simulink model "Bilanciamento_MPC_2024b"  (R2024b)
settings: Solver=FixedStepDiscrete  StartTime=0  StopTime=par_sim.t_fine  FixedStep=par_sim.Tint  RelTol=1e-3
PostLoadFcn:
  | % Path: la cartella di questo modello e le cartelle del progetto
  | % MPC_Range_Extension, due livelli sopra. La cartella del modello si
  | % aggiunge per ultima, cosi' ha la precedenza su altre versioni (v1.0).
  | cartella_modello  = fileparts(get_param('Bilanciamento_MPC', 'FileName'));
  | cartella_progetto = fileparts(fileparts(cartella_modello));
  | addpath(cartella_progetto, fullfile(cartella_progetto, 'modello'), fullfile(cartella_progetto, 'mpc'), fullfile(cartella_progetto, 'simulazione'), fullfile(cartella_progetto, 'grafici'));
  | addpath(cartella_modello);
  | clear cartella_modello cartella_progetto
  | 
  | % Parametri della simulazione, se non ci sono gia' (parametri_simulazione.m)
  | if ~evalin('base', 'exist(''par_sim'', ''var'')')
  |     assignin('base', 'par_sim', parametri_simulazione());
  | end
InitFcn:
  | % Path: la cartella di questo modello e le cartelle del progetto
  | % MPC_Range_Extension, due livelli sopra. La cartella del modello si
  | % aggiunge per ultima, cosi' ha la precedenza su altre versioni (v1.0).
  | cartella_modello  = fileparts(get_param('Bilanciamento_MPC', 'FileName'));
  | cartella_progetto = fileparts(fileparts(cartella_modello));
  | addpath(cartella_progetto, fullfile(cartella_progetto, 'modello'), fullfile(cartella_progetto, 'mpc'), fullfile(cartella_progetto, 'simulazione'), fullfile(cartella_progetto, 'grafici'));
  | addpath(cartella_modello);
  | clear cartella_modello cartella_progetto
  | 
  | % Parametri della simulazione, se non ci sono gia' (parametri_simulazione.m)
  | if ~evalin('base', 'exist(''par_sim'', ''var'')')
  |     assignin('base', 'par_sim', parametri_simulazione());
  | end
values from neighbouring files (symbols this model uses):
  par_sim = parametri_simulazione(par, pacco, formulazione, par.(['scenario' scenario]), orizzonte)    [avvio_simulink.m]    (also in simula_simulink.m = parametri_simulazione(par, pacco, tipo, scen, p))
libraries: simulink x2
settings Model: Creator=Acer  LastModifiedBy=Acer
settings ModelReferenceCC: UpdateModelReferenceTargets=IfOutOfDate
settings SFSimCC: SimGPUStackLimitPerThread=51200
settings RTWCC: GPUStackLimitPerThread=51200  GPUComputeCapability=7.5
settings ConfigComp: CovMetricSettings=de  CovBoundaryAbsTol=1.0e-5

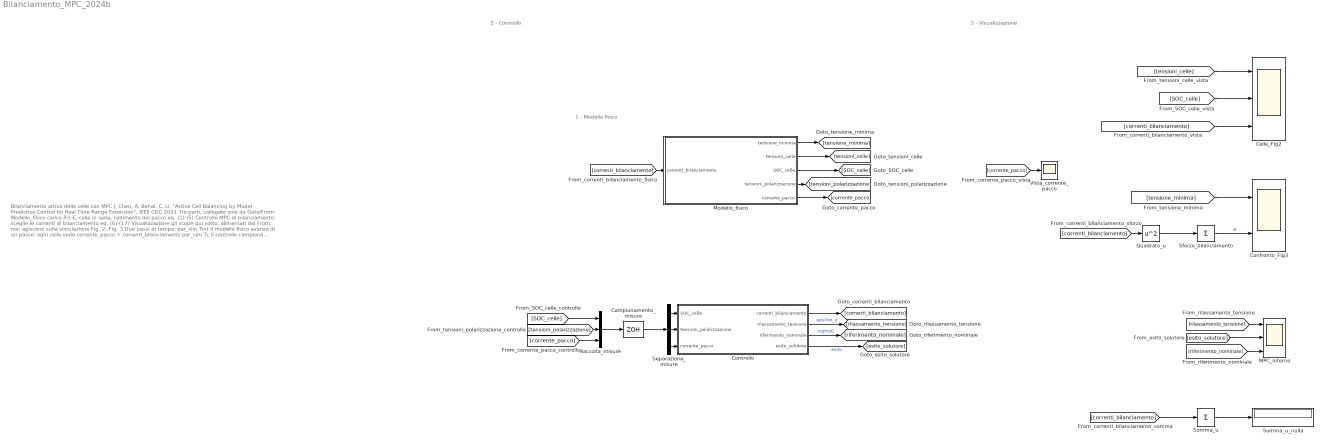
== system Bilanciamento_MPC_2024b ==
  note: Bilanciamento attivo delle celle con MPC
      | J. Chen, A. Behal, C. Li, "Active Cell Balancing by Model Predictive Control for Real Time Range Extension", IEEE CDC 2021
      |
      | Tre parti, collegate solo da Goto/From:
      |    Modello_fisico     carico R-L-E, celle in serie, cedimento del pacco             eq. (1)-(5)
      |    Controllo          MPC di bilanciamento: sceglie le correnti di bilanciamento    eq. (6)-(17)
      |    Visualizzazione    gli scope qui sotto, alimentati dai From: non agiscono sulla simulazione   Fig. 2, Fig. 3
      |
      | Due passi di tempo:
      |    par_sim.Tint         il modello fisico avanza di un passo: ogni cella vede corrente_pacco + correnti_bilanciamento
      |    par_sim.Tc           il controllo campiona corrente_pacco, SOC_celle e tensioni_polarizzazione e sceglie correnti_bilanciamento,
      |                         che restano costanti fino al passo di controllo successivo
      | La simulazione si ferma quando una cella scende sotto y_min.
      |
      | Parametri della simulazione nella struct 'par_sim' (avvio_simulink.m).
      | par_sim.n_J: 1 = J_t   2 = J_m   3 = J_Delta.  Confronto dei quattro casi: main_simulink.m
  note: 1 - Modello fisico
  note: 2 - Controllo
  note: 3 - Visualizzazione
  Campionamento_misure : ZeroOrderHold  SampleTime=par_sim.Tc
      settings: AttributesFormatString=ogni Tc
  Celle_Fig2 : Scope  NumInputPorts=3
      settings: AttributesFormatString=Fig. 2: y, s, u
  Confronto_Fig3 : Scope  NumInputPorts=2
      settings: AttributesFormatString=Fig. 3: min y, sforzo w
  Controllo : Subsystem
      settings: AttributesFormatString=MPC: problema (6) risolto\ncome QP (Remark 3)
  MPC_interno : Scope  NumInputPorts=3
      settings: AttributesFormatString=epsilon_y, esito, sigma0
  Modello_fisico : Subsystem
      settings: AttributesFormatString=carico, celle, cedimento\neq. (1)-(5)
  Quadrato_u : Math  Operator=square
  Raccolta_misure : Mux  Inputs=[par_sim.N par_sim.N 1]
  Separazione_misure : Demux  Outputs=[par_sim.N par_sim.N 1]
  Sforzo_bilanciamento : Sum  Inputs=+
  Somma_u : Sum  Inputs=+
      settings: AttributesFormatString=eq. (6f)
  Somma_u_nulla : Display
      settings: AttributesFormatString=deve restare 0
  Vista_corrente_pacco : Scope
  wires:
  [correnti_bilanciamento] -> Quadrato_u/1
  Quadrato_u/1 -> Sforzo_bilanciamento/1
  [correnti_bilanciamento] -> Somma_u/1
  [correnti_bilanciamento] -> Celle_Fig2/3
  [riferimento_nominale] -> MPC_interno/3
  [esito_solutore] -> MPC_interno/2
  [SOC_celle] -> Celle_Fig2/2
  [rilassamento_tensione] -> MPC_interno/1
  [tensioni_celle] -> Celle_Fig2/1
  Sforzo_bilanciamento/1 -> Confronto_Fig3/2  "w"
  [tensione_minima] -> Confronto_Fig3/1
  Somma_u/1 -> Somma_u_nulla/1
  Controllo/4(esito_solutore) -> [esito_solutore]  "esito"
  Controllo/3(riferimento_nominale) -> [riferimento_nominale]  "sigma0"
  Controllo/2(rilassamento_tensione) -> [rilassamento_tensione]  "epsilon_y"
  Controllo/1(correnti_bilanciamento) -> [correnti_bilanciamento]
  Modello_fisico/5(corrente_pacco) -> [corrente_pacco]
  Modello_fisico/4(tensioni_polarizzazione) -> [tensioni_polarizzazione]
  Modello_fisico/3(SOC_celle) -> [SOC_celle]
  Modello_fisico/2(tensioni_celle) -> [tensioni_celle]
  Modello_fisico/1(tensione_minima) -> [tensione_minima]
  [correnti_bilanciamento] -> Modello_fisico/1(correnti_bilanciamento)
  [corrente_pacco] -> Vista_corrente_pacco/1
  [tensioni_polarizzazione] -> Raccolta_misure/2
  [SOC_celle] -> Raccolta_misure/1
  [corrente_pacco] -> Raccolta_misure/3
  Raccolta_misure/1 -> Campionamento_misure/1
  Campionamento_misure/1 -> Separazione_misure/1
  Separazione_misure/3 -> Controllo/3(corrente_pacco)
  Separazione_misure/2 -> Controllo/2(tensioni_polarizzazione)
  Separazione_misure/1 -> Controllo/1(SOC_celle)

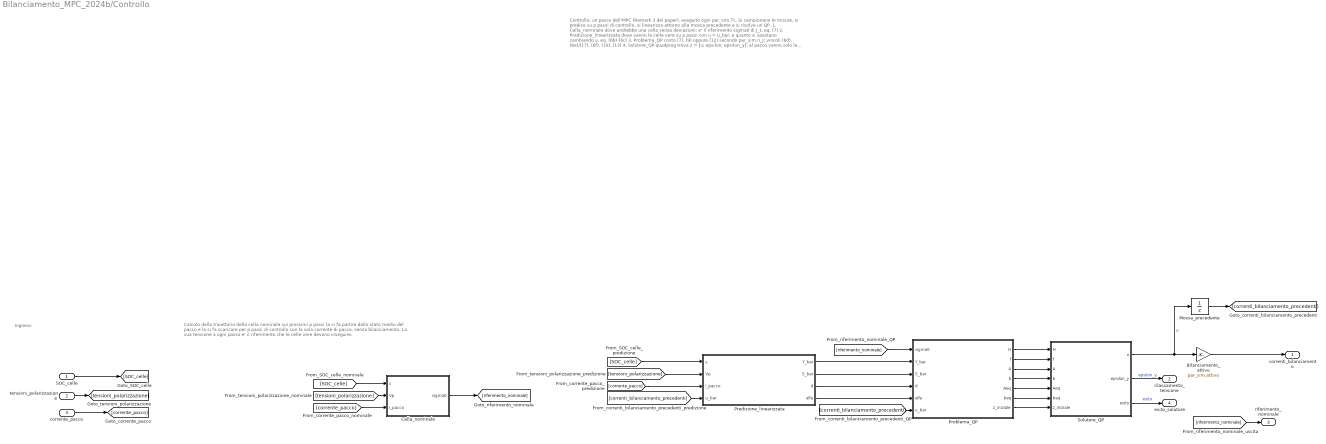
== system Bilanciamento_MPC_2024b/Controllo ==
  note: Ingressi
  note: Calcolo della traiettoria della cella nominale sui prossimi p passi
      |
      | la si fa partire dallo stato medio del pacco e la si fa scaricare per p passi di controllo con la sola corrente di pacco, senza bilanciamento.
      | La sua tensione a ogni passo e' il riferimento che le celle vere devono inseguire.
  note: Controllo: un passo dell'MPC (Remark 3 del paper), eseguito ogni par_sim.Tc. Si campionano le misure, si predice su p passi di controllo,
      | si linearizza attorno alla mossa precedente e si risolve un QP.
      |
      | 1. Cella_nominale            dove andrebbe una cella senza deviazioni: e' il riferimento sigma0 di J_t, eq. (7)
      | 2. Predizione_linearizzata   dove vanno le celle vere su p passi con u = u_bar, e quanto si spostano cambiando u, eq. (6b)-(6c)
      | 3. Problema_QP               costo (7), (9) oppure (12) secondo par_sim.n_J; vincoli (6d), (6e)/(17), (6f), (10), (13)
      | 4. Solutore_QP               quadprog trova z = [u; epsilon; epsilon_y]; al pacco vanno solo le u (orizzonte mobile)
      | 5. Bilanciamento_attivo      guadagno par_sim.attivo: con 0 il pacco lavora senza bilanciamento
      |
      | Doppio clic su un blocco per leggerne il codice: il calcolo e' tutto dentro il blocco.
  SOC_celle : Inport
  tensioni_polarizzazione : Inport  Port=2
  corrente_pacco : Inport  Port=3
  Bilanciamento_attivo : Gain  Gain=par_sim.attivo
      settings: AttributesFormatString=par_sim.attivo: 0 o 1
  Cella_nominale : MATLAB Function  TreatAsAtomicUnit=on
      settings: AttributesFormatString=eq. (7): riferimento sigma0
  Mossa_precedente : UnitDelay  InitialCondition=zeros(par_sim.N, 1)  SampleTime=par_sim.Tc
      settings: AttributesFormatString=u_bar = u_(k-1)
  Predizione_linearizzata : MATLAB Function  TreatAsAtomicUnit=on
      settings: AttributesFormatString=eq. (6b)-(6c), Remark 3
  Problema_QP : MATLAB Function  TreatAsAtomicUnit=on
      settings: AttributesFormatString=costo (7)/(9)/(12) e vincoli
  Solutore_QP : MATLAB Function  TreatAsAtomicUnit=on
      settings: AttributesFormatString=quadprog
  correnti_bilanciamento : Outport
  rilassamento_tensione : Outport  Port=2
  riferimento_nominale : Outport  Port=3
  esito_solutore : Outport  Port=4
  wires:
  corrente_pacco/1 -> [corrente_pacco]
  [corrente_pacco] -> Predizione_linearizzata/3(i_pacco)
  [tensioni_polarizzazione] -> Predizione_linearizzata/2(Vp)
  [SOC_celle] -> Predizione_linearizzata/1(s)
  [corrente_pacco] -> Cella_nominale/3(i_pacco)
  [tensioni_polarizzazione] -> Cella_nominale/2(Vp)
  [SOC_celle] -> Cella_nominale/1(s)
  Cella_nominale/1(sigma0) -> [riferimento_nominale]
  Predizione_linearizzata/1(Y_bar) -> Problema_QP/2(Y_bar)
  Predizione_linearizzata/2(S_bar) -> Problema_QP/3(S_bar)
  Predizione_linearizzata/3(d) -> Problema_QP/4(d)
  Predizione_linearizzata/4(alfa) -> Problema_QP/5(alfa)
  Problema_QP/1(H) -> Solutore_QP/1(H)
  Problema_QP/2(f) -> Solutore_QP/2(f)
  Problema_QP/3(A) -> Solutore_QP/3(A)
  Problema_QP/4(b) -> Solutore_QP/4(b)
  Problema_QP/5(Aeq) -> Solutore_QP/5(Aeq)
  Problema_QP/6(beq) -> Solutore_QP/6(beq)
  Problema_QP/7(z_iniziale) -> Solutore_QP/7(z_iniziale)
  [correnti_bilanciamento_precedenti] -> Predizione_linearizzata/4(u_bar)
  [correnti_bilanciamento_precedenti] -> Problema_QP/6(u_bar)
  Mossa_precedente/1 -> [correnti_bilanciamento_precedenti]
  Bilanciamento_attivo/1 -> correnti_bilanciamento/1
  Solutore_QP/1(u) -> Mossa_precedente/1, Bilanciamento_attivo/1  "u"
  tensioni_polarizzazione/1 -> [tensioni_polarizzazione]
  SOC_celle/1 -> [SOC_celle]
  [riferimento_nominale] -> riferimento_nominale/1
  [riferimento_nominale] -> Problema_QP/1(sigma0)
  Solutore_QP/2(epsilon_y) -> rilassamento_tensione/1  "epsilon_y"
  Solutore_QP/3(esito) -> esito_solutore/1  "esito"

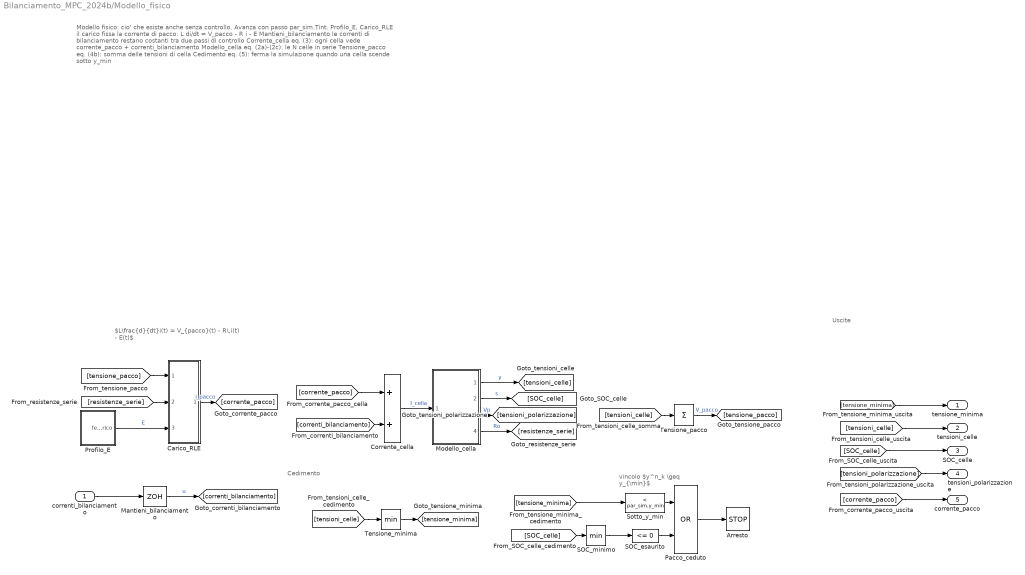
== system Bilanciamento_MPC_2024b/Modello_fisico ==
  note: vincolo $y^n_k \geq y_{\min}$
  note: $L\frac{d}{dt}i(t) = V_{pacco}(t) - R\,i(t) - E(t)$
  note: Cedimento
  note: Uscite
  note: Modello fisico: cio' che esiste anche senza controllo. Avanza con passo par_sim.Tint.
      |
      |    Profilo_E, Carico_RLE   il carico fissa la corrente di pacco:  L di/dt = V_pacco - R i - E
      |    Mantieni_bilanciamento  le correnti di bilanciamento restano costanti tra due passi di controllo
      |    Corrente_cella          eq. (3): ogni cella vede corrente_pacco + correnti_bilanciamento
      |    Modello_cella           eq. (2a)-(2c): le N celle in serie
      |    Tensione_pacco          eq. (4b): somma delle tensioni di cella
      |    Cedimento               eq. (5): ferma la simulazione quando una cella scende sotto y_min
  correnti_bilanciamento : Inport
  Arresto : Stop
  Carico_RLE : Subsystem
      settings: AttributesFormatString=L di_pacco/dt = V_pacco - R i_pacco - E
  Corrente_cella : Sum
      settings: AttributesFormatString=eq. (3): I_cella = i_pacco + u
  Mantieni_bilanciamento : ZeroOrderHold  SampleTime=par_sim.Tint
      settings: AttributesFormatString=costante tra due passi\ndi controllo
  Modello_cella : Subsystem
      settings: AttributesFormatString=eq. (2a)-(2c), (4a)
  Pacco_ceduto : Logic  Operator=OR  AllPortsSameDT=off  OutDataTypeStr=boolean
  Profilo_E : Subsystem
      settings: AttributesFormatString=f.e.m. del carico E(t)
  SOC_esaurito : simulink/Logic and Bit Operations/Compare To Constant  relop=<=  const=0  OutDataTypeStr=boolean
  SOC_minimo : MinMax
  Sotto_y_min : simulink/Logic and Bit Operations/Compare To Constant  relop=<  const=par_sim.y_min  OutDataTypeStr=boolean
  Tensione_minima : MinMax
  Tensione_pacco : Sum  Inputs=+
      settings: AttributesFormatString=eq. (4b)
  tensione_minima : Outport
  tensioni_celle : Outport  Port=2
  SOC_celle : Outport  Port=3
  tensioni_polarizzazione : Outport  Port=4
  corrente_pacco : Outport  Port=5
  wires:
  correnti_bilanciamento/1 -> Mantieni_bilanciamento/1
  [tensioni_celle] -> Tensione_pacco/1
  Modello_cella/1(tensioni_celle) -> [tensioni_celle]  "y"
  [correnti_bilanciamento] -> Corrente_cella/2
  [tensione_pacco] -> Carico_RLE/1(tensione_pacco)
  Modello_cella/2(SOC_celle) -> [SOC_celle]  "s"
  Tensione_pacco/1 -> [tensione_pacco]  "V_pacco"
  [resistenze_serie] -> Carico_RLE/2(resistenze_serie)
  Modello_cella/4(resistenze_serie) -> [resistenze_serie]  "Ro"
  Profilo_E/1(fem_carico) -> Carico_RLE/3(fem_carico)  "E"
  Corrente_cella/1 -> Modello_cella/1(correnti_celle)  "I_cella"
  Carico_RLE/1(corrente_pacco) -> [corrente_pacco]  "i_pacco"
  [corrente_pacco] -> Corrente_cella/1
  Mantieni_bilanciamento/1 -> [correnti_bilanciamento]  "u"
  [corrente_pacco] -> corrente_pacco/1
  [tensione_minima] -> tensione_minima/1
  [SOC_celle] -> SOC_celle/1
  Modello_cella/3(tensioni_polarizzazione) -> [tensioni_polarizzazione]  "Vp"
  [tensioni_polarizzazione] -> tensioni_polarizzazione/1
  [tensioni_celle] -> tensioni_celle/1
  Sotto_y_min/1 -> Pacco_ceduto/1
  [tensione_minima] -> Sotto_y_min/1
  SOC_minimo/1 -> SOC_esaurito/1
  Pacco_ceduto/1 -> Arresto/1
  [SOC_celle] -> SOC_minimo/1
  SOC_esaurito/1 -> Pacco_ceduto/2
  [tensioni_celle] -> Tensione_minima/1
  Tensione_minima/1 -> [tensione_minima]

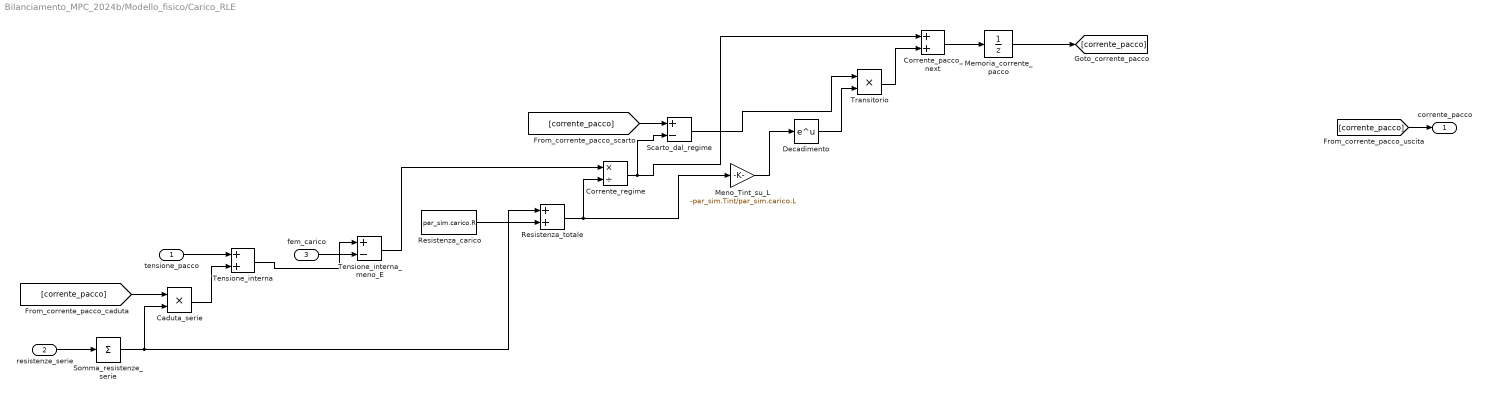
== system Bilanciamento_MPC_2024b/Modello_fisico/Carico_RLE ==
  tensione_pacco : Inport
  resistenze_serie : Inport  Port=2
  fem_carico : Inport  Port=3
  Caduta_serie : Product  Inputs=**
  Corrente_pacco_next : Sum
  Corrente_regime : Product  Inputs=*/
      settings: AttributesFormatString=(V_int - E) / R_tot
  Decadimento : Math
      settings: AttributesFormatString=exp(-Tint*R_tot/L)
  Memoria_corrente_pacco : UnitDelay  InitialCondition=par_sim.i_pacco_iniziale  SampleTime=par_sim.Tint
      settings: AttributesFormatString=stato i_pacco
  Meno_Tint_su_L : Gain  Gain=-par_sim.Tint/par_sim.carico.L
  Resistenza_carico : Constant  Value=par_sim.carico.R  SampleTime=par_sim.Tint
  Resistenza_totale : Sum
  Scarto_dal_regime : Sum  Inputs=+-
  Somma_resistenze_serie : Sum  Inputs=+
  Tensione_interna : Sum
      settings: AttributesFormatString=tensione del pacco a i_pacco = 0
  Tensione_interna_meno_E : Sum  Inputs=+-
  Transitorio : Product  Inputs=**
  corrente_pacco : Outport
  wires:
  [corrente_pacco] -> Scarto_dal_regime/1
  [corrente_pacco] -> Caduta_serie/1
  resistenze_serie/1 -> Somma_resistenze_serie/1
  Somma_resistenze_serie/1 -> Caduta_serie/2, Resistenza_totale/1
  Resistenza_carico/1 -> Resistenza_totale/2
  Memoria_corrente_pacco/1 -> [corrente_pacco]
  tensione_pacco/1 -> Tensione_interna/1
  Caduta_serie/1 -> Tensione_interna/2
  Tensione_interna/1 -> Tensione_interna_meno_E/1
  fem_carico/1 -> Tensione_interna_meno_E/2
  Tensione_interna_meno_E/1 -> Corrente_regime/1
  Resistenza_totale/1 -> Meno_Tint_su_L/1, Corrente_regime/2
  Meno_Tint_su_L/1 -> Decadimento/1
  Corrente_regime/1 -> Corrente_pacco_next/1, Scarto_dal_regime/2
  Scarto_dal_regime/1 -> Transitorio/1
  Decadimento/1 -> Transitorio/2
  Transitorio/1 -> Corrente_pacco_next/2
  Corrente_pacco_next/1 -> Memoria_corrente_pacco/1
  [corrente_pacco] -> corrente_pacco/1

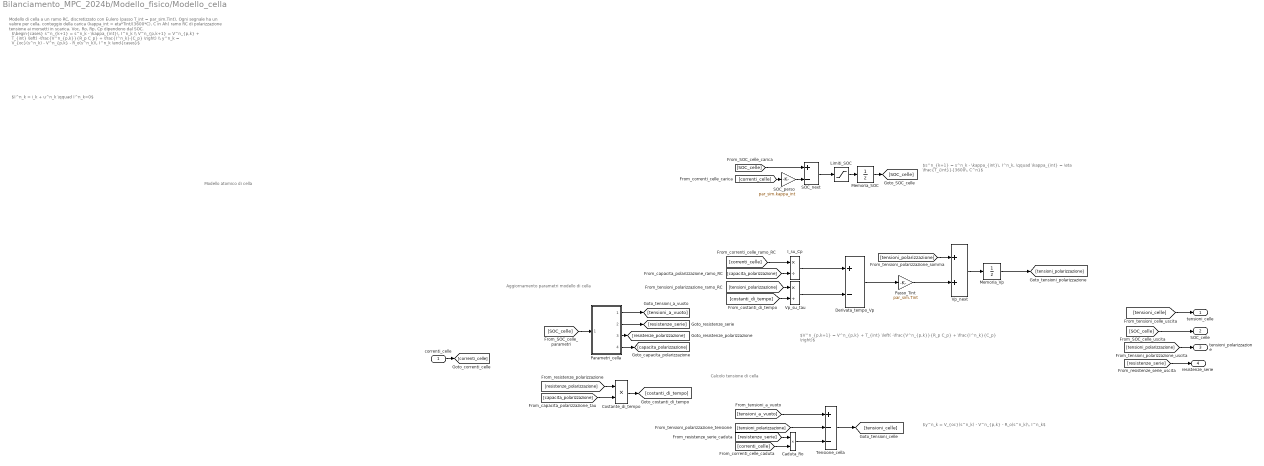
== system Bilanciamento_MPC_2024b/Modello_fisico/Modello_cella ==
  note: Modello atomico di cella
  note: $I^n_k = i_k + u^n_k \qquad I^n_k>0$
  note: $\begin{cases} s^n_{k+1} = s^n_k - \kappa_{int}\, I^n_k \\ V^n_{p,k+1} = V^n_{p,k} + T_{int} \left( -\frac{V^n_{p,k}}{R_p C_p} + \frac{I^n_k}{C_p} \right) \\ y^n_k = V_{oc}(s^n_k) - V^n_{p,k} - R_o(s^n_k)\, I^n_k \end{cases}$
  note: Calcolo tensione di cella
  note: Aggiornamento parametri modello di cella
  note: Modello di cella a un ramo RC, discretizzato con Eulero (passo T_int = par_sim.Tint). Ogni segnale ha un valore per cella.
      |
      | conteggio della carica (kappa_int = eta*Tint/(3600*C), C in Ah)
      |
      | ramo RC di polarizzazione
      |
      | tensione ai morsetti
      |
      | in scarica. Voc, Ro, Rp, Cp dipendono dal SOC.
  note: $V^n_{p,k+1} = V^n_{p,k} + T_{int} \left( -\frac{V^n_{p,k}}{R_p C_p} + \frac{I^n_k}{C_p} \right)$
  note: $y^n_k = V_{oc}(s^n_k) - V^n_{p,k} - R_o(s^n_k)\, I^n_k$
  note: $s^n_{k+1} = s^n_k - \kappa_{int}\, I^n_k, \qquad \kappa_{int} = \eta \frac{T_{int}}{3600\, C^n}$
  correnti_celle : Inport
  Caduta_Ro : Product  Inputs=**
  Costante_di_tempo : Product  Inputs=**
  Derivata_tempo_Vp : Sum  Inputs=+-
  I_su_Cp : Product  Inputs=*/
  Limiti_SOC : Saturate  UpperLimit=1  LowerLimit=0
  Memoria_SOC : UnitDelay  InitialCondition=par_sim.s_iniziale  SampleTime=par_sim.Tint
      settings: AttributesFormatString=stato s
  Memoria_Vp : UnitDelay  InitialCondition=par_sim.Vp_iniziale  SampleTime=par_sim.Tint
      settings: AttributesFormatString=stato V_p
  Parametri_cella : Subsystem
      settings: AttributesFormatString=V_oc, R_o, R_p, C_p(SOC)
  Passo_Tint : Gain  Gain=par_sim.Tint
  SOC_next : Sum  Inputs=+-
  SOC_perso : Gain  Gain=par_sim.kappa_int
      settings: AttributesFormatString=kappa_int * I_cella
  Tensione_cella : Sum  Inputs=+--
      settings: AttributesFormatString=eq. (2c)
  Vp_next : Sum
      settings: AttributesFormatString=eq. (2b)
  Vp_su_tau : Product  Inputs=*/
  tensioni_celle : Outport
  SOC_celle : Outport  Port=2
  tensioni_polarizzazione : Outport  Port=3
  resistenze_serie : Outport  Port=4
  wires:
  correnti_celle/1 -> [correnti_celle]
  [tensioni_polarizzazione] -> Vp_next/1
  [tensioni_polarizzazione] -> Vp_su_tau/1
  [tensioni_polarizzazione] -> Tensione_cella/2
  [SOC_celle] -> SOC_celle/1
  [SOC_celle] -> SOC_next/1
  [correnti_celle] -> I_su_Cp/1
  [correnti_celle] -> SOC_perso/1
  [correnti_celle] -> Caduta_Ro/2
  Vp_next/1 -> Memoria_Vp/1
  Passo_Tint/1 -> Vp_next/2
  Derivata_tempo_Vp/1 -> Passo_Tint/1
  Vp_su_tau/1 -> Derivata_tempo_Vp/2
  I_su_Cp/1 -> Derivata_tempo_Vp/1
  Limiti_SOC/1 -> Memoria_SOC/1
  SOC_next/1 -> Limiti_SOC/1
  SOC_perso/1 -> SOC_next/2
  Caduta_Ro/1 -> Tensione_cella/3
  Memoria_Vp/1 -> [tensioni_polarizzazione]
  Memoria_SOC/1 -> [SOC_celle]
  [SOC_celle] -> Parametri_cella/1(SOC_celle)
  [resistenze_serie] -> resistenze_serie/1
  [resistenze_serie] -> Caduta_Ro/1
  Parametri_cella/2(resistenze_serie) -> [resistenze_serie]
  [resistenze_polarizzazione] -> Costante_di_tempo/1
  Parametri_cella/3(resistenze_polarizzazione) -> [resistenze_polarizzazione]
  Parametri_cella/4(capacita_polarizzazione) -> [capacita_polarizzazione]
  [capacita_polarizzazione] -> Costante_di_tempo/2
  [capacita_polarizzazione] -> I_su_Cp/2
  [tensioni_a_vuoto] -> Tensione_cella/1
  Parametri_cella/1(tensioni_a_vuoto) -> [tensioni_a_vuoto]
  Costante_di_tempo/1 -> [costanti_di_tempo]
  [costanti_di_tempo] -> Vp_su_tau/2
  [tensioni_polarizzazione] -> tensioni_polarizzazione/1
  [tensioni_celle] -> tensioni_celle/1
  Tensione_cella/1 -> [tensioni_celle]

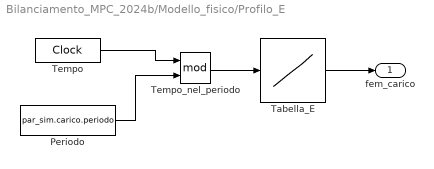
== system Bilanciamento_MPC_2024b/Modello_fisico/Profilo_E ==
  Periodo : Constant  Value=par_sim.carico.periodo  SampleTime=par_sim.Tint
  Tabella_E : Lookup_n-D  NumberOfTableDimensions=1  BreakpointsForDimension1=par_sim.carico.t_E  Table=par_sim.carico.E  ExtrapMethod=Clip  InternalRulePriority=Speed  RndMeth=Simplest
  Tempo : DigitalClock  SampleTime=par_sim.Tint
  Tempo_nel_periodo : Math  Operator=mod
  fem_carico : Outport
  wires:
  Tempo/1 -> Tempo_nel_periodo/1
  Periodo/1 -> Tempo_nel_periodo/2
  Tempo_nel_periodo/1 -> Tabella_E/1
  Tabella_E/1 -> fem_carico/1

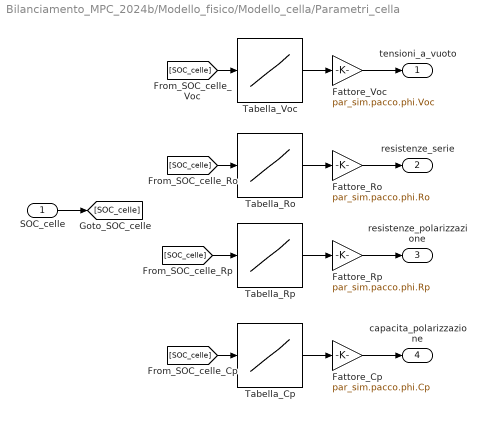
== system Bilanciamento_MPC_2024b/Modello_fisico/Modello_cella/Parametri_cella ==
  SOC_celle : Inport
  Fattore_Cp : Gain  Gain=par_sim.pacco.phi.Cp
  Fattore_Ro : Gain  Gain=par_sim.pacco.phi.Ro
  Fattore_Rp : Gain  Gain=par_sim.pacco.phi.Rp
  Fattore_Voc : Gain  Gain=par_sim.pacco.phi.Voc
  Tabella_Cp : Lookup_n-D  NumberOfTableDimensions=1  BreakpointsForDimension1=par_sim.pacco.s_tab  Table=par_sim.pacco.Cp_tab  ExtrapMethod=Clip  InternalRulePriority=Speed  RndMeth=Simplest
  Tabella_Ro : Lookup_n-D  NumberOfTableDimensions=1  BreakpointsForDimension1=par_sim.pacco.s_tab  Table=par_sim.pacco.Ro_tab  ExtrapMethod=Clip  InternalRulePriority=Speed  RndMeth=Simplest
  Tabella_Rp : Lookup_n-D  NumberOfTableDimensions=1  BreakpointsForDimension1=par_sim.pacco.s_tab  Table=par_sim.pacco.Rp_tab  ExtrapMethod=Clip  InternalRulePriority=Speed  RndMeth=Simplest
  Tabella_Voc : Lookup_n-D  NumberOfTableDimensions=1  BreakpointsForDimension1=par_sim.pacco.s_tab  Table=par_sim.pacco.Voc_tab  ExtrapMethod=Clip  InternalRulePriority=Speed  RndMeth=Simplest
  tensioni_a_vuoto : Outport
  resistenze_serie : Outport  Port=2
  resistenze_polarizzazione : Outport  Port=3
  capacita_polarizzazione : Outport  Port=4
  wires:
  Tabella_Voc/1 -> Fattore_Voc/1
  Tabella_Ro/1 -> Fattore_Ro/1
  Tabella_Rp/1 -> Fattore_Rp/1
  Tabella_Cp/1 -> Fattore_Cp/1
  Fattore_Voc/1 -> tensioni_a_vuoto/1
  Fattore_Ro/1 -> resistenze_serie/1
  Fattore_Rp/1 -> resistenze_polarizzazione/1
  Fattore_Cp/1 -> capacita_polarizzazione/1
  SOC_celle/1 -> [SOC_celle]
  [SOC_celle] -> Tabella_Rp/1
  [SOC_celle] -> Tabella_Cp/1
  [SOC_celle] -> Tabella_Voc/1
  [SOC_celle] -> Tabella_Ro/1

== matlab function Bilanciamento_MPC_2024b/Controllo/Predizione_linearizzata ==
  data: s input; Y_bar output; Vp input; i_pacco input; u_bar input; S_bar output; d output; alfa output; par_sim parameter
function [Y_bar, S_bar, d, alfa] = Predizione_linearizzata(s, Vp, i_pacco, u_bar, par_sim)
% PREDIZIONE LINEARIZZATA - eq. (6b)-(6c) del paper, linearizzate come nel
% Remark 3.
%
% Per ogni cella fa avanzare il modello per p passi di controllo, con la
% corrente di bilanciamento del passo precedente, e accanto a ogni
% equazione del modello calcola la sua derivata rispetto alla corrente.
% Con questi numeri la tensione e il SOC predetti diventano due rette
% nella corrente di bilanciamento u(n), [L, (6)]:
%
%   y(j,n) ~= Y_bar(j,n) + d(j,n)    * (u(n) - u_bar(n))
%   s(j,n) ~= S_bar(j,n) + alfa(j,n) * (u(n) - u_bar(n))
%
% Ingressi, all'istante k
%   s, Vp     SOC e tensione di polarizzazione misurati, N x 1
%   i_pacco   corrente di pacco misurata [A], positiva in scarica
%   u_bar     correnti di bilanciamento del passo precedente, N x 1
%   par_sim   parametri della simulazione (parametri_simulazione.m)
% Uscite, matrici p x N: riga j <-> istante k+j, colonna n <-> cella n
%   Y_bar, S_bar   tensione e SOC predetti con u = u_bar
%   d, alfa        coefficienti di sensibilita': di quanto cambiano la
%                  tensione [V/A] e il SOC [1/A] per ogni ampere in piu'
%
% Formule e numeri di equazione: Linearizzazione_MPC.pdf, citato [L].
% Le celle non si influenzano tra loro: si calcola una cella alla volta.

%% Dati
N  = par_sim.N;                         % numero di celle
p  = par_sim.p;                         % passi dell'orizzonte
Tc = par_sim.Tc;                        % [s] passo di controllo

% Tabelle nominali: ogni parametro in 7 punti di SOC, [L, sezione 2.2]
s_tab   = par_sim.pacco.s_tab;
Voc_tab = par_sim.pacco.Voc_tab;        % [V]   tensione a vuoto
Ro_tab  = par_sim.pacco.Ro_tab;         % [Ohm] resistenza serie
Rp_tab  = par_sim.pacco.Rp_tab;         % [Ohm] resistenza di polarizzazione
Cp_tab  = par_sim.pacco.Cp_tab;         % [F]   capacita' di polarizzazione

Y_bar = zeros(p, N);
S_bar = zeros(p, N);
d     = zeros(p, N);
alfa  = zeros(p, N);

%% Una cella alla volta
for n = 1:N

    % Parametri propri della cella n: ogni parametro e' la tabella nominale
    % per il fattore di deviazione phi della cella; kappa e' il SOC perso
    % in un passo per ogni ampere, [L, (5)]
    phi_Voc = par_sim.pacco.phi.Voc(n);
    phi_Ro  = par_sim.pacco.phi.Ro(n);
    phi_Rp  = par_sim.pacco.phi.Rp(n);
    phi_Cp  = par_sim.pacco.phi.Cp(n);
    kappa   = par_sim.pacco.kappa(n);

    % Punto di partenza: lo stato misurato. s_j e Vp_j contengono lo stato
    % della cella e vengono aggiornati a ogni passo: prima dell'aggiornamento
    % valgono all'istante k+j-1, dopo all'istante k+j.
    s_j  = s(n);
    Vp_j = Vp(n);

    % Corrente della cella nel punto di linearizzazione, costante su tutto
    % l'orizzonte, [L, (1)]
    I_cella = i_pacco + u_bar(n);

    % Derivate dello stato rispetto alla corrente: nulle all'istante k,
    % perche' lo stato misurato non dipende dalla corrente futura
    alfa_j = 0;                         % derivata del SOC
    beta_j = 0;                         % derivata della tensione di polarizzazione

    %% Un passo alla volta
    for j = 1:p

        % 1) Parametri del ramo RC e loro derivate rispetto al SOC, letti nel
        %    SOC di inizio passo
        [Rp, ds_Rp] = leggi_tabella(s_tab, Rp_tab, phi_Rp, s_j);
        [Cp, ds_Cp] = leggi_tabella(s_tab, Cp_tab, phi_Cp, s_j);
        tau    = Rp * Cp;                       % costante di tempo
        ds_tau = ds_Rp * Cp + Rp * ds_Cp;       % sua derivata rispetto al SOC

        % 2) Tensione di polarizzazione, [L, (3)], e sua derivata, [L, (7)].
        %    beta_j si aggiorna per prima, perche' usa Vp_j e alfa_j di
        %    inizio passo.
        beta_j = beta_j + Tc * ( -beta_j / tau ...                      % Vp dipende dalla corrente
                                 + Vp_j * ds_tau * alfa_j / tau^2 ...   % tau tramite il SOC
                                 + 1 / Cp ...                           % corrente diretta
                                 - I_cella * ds_Cp * alfa_j / Cp^2 );   % Cp tramite il SOC
        Vp_j   = Vp_j + Tc * (-Vp_j / tau + I_cella / Cp);

        % 3) SOC, [L, (2)], e sua derivata, [L, (8)]
        s_j    = s_j - kappa * I_cella;
        alfa_j = alfa_j - kappa;
        if s_j >= 1                     % una cella piena non si carica oltre
            s_j    = 1;
            alfa_j = 0;
        end

        % 4) Tensione ai morsetti, [L, (4)], e sua derivata, [L, (9)], con i
        %    parametri letti nel SOC di fine passo
        [Voc, ds_Voc] = leggi_tabella(s_tab, Voc_tab, phi_Voc, s_j);
        [Ro,  ds_Ro]  = leggi_tabella(s_tab, Ro_tab,  phi_Ro,  s_j);
        y   = Voc - Vp_j - Ro * I_cella;
        d_j = ds_Voc * alfa_j ...                   % Voc tramite il SOC
              - beta_j ...                          % Vp dipende dalla corrente
              - ds_Ro * alfa_j * I_cella ...        % Ro tramite il SOC
              - Ro;                                 % corrente diretta

        % 5) Riga j, colonna n delle quattro uscite
        Y_bar(j, n) = y;
        S_bar(j, n) = s_j;
        d(j, n)     = d_j;
        alfa(j, n)  = alfa_j;

    end
end

end


function [P, ds_P] = leggi_tabella(s_tab, P_tab, phi, s)
% Valore del parametro P nel SOC s e sua derivata rispetto al SOC, [L, (T)]:
%
%   P(s) = phi * ( P_tab(tratto) + m * (s - s_tab(tratto)) ),   ds_P = phi * m
%
% dove tratto e' il tratto della tabella che contiene s e m la sua
% pendenza. Fuori dalla tabella si usa il valore dell'estremo, con derivata
% nulla.

% SOC riportato dentro la tabella
s_limitato = min(max(s, s_tab(1)), s_tab(end));

% Tratto della tabella: s_tab(tratto) <= s_limitato < s_tab(tratto + 1).
% L'ultimo punto della tabella appartiene all'ultimo tratto.
tratto = 1;
for q = 2:numel(s_tab) - 1
    if s_limitato >= s_tab(q)
        tratto = q;
    end
end

% Pendenza del tratto, valore e derivata
m    = (P_tab(tratto + 1) - P_tab(tratto)) / (s_tab(tratto + 1) - s_tab(tratto));
P    = phi * (P_tab(tratto) + m * (s_limitato - s_tab(tratto)));
ds_P = phi * m;

if s < s_tab(1) || s > s_tab(end)       % fuori dalla tabella
    ds_P = 0;
end

end

== matlab function Bilanciamento_MPC_2024b/Controllo/Cella_nominale ==
  data: s input; sigma0 output; Vp input; i_pacco input; par_sim parameter
function sigma0 = Cella_nominale(s, Vp, i_pacco, par_sim)
% CELLA NOMINALE - riferimento sigma0 del costo J_t, eq. (7) del paper.
%
% Si prende una cella "ideale", con i parametri nominali (senza deviazioni),
% la si fa partire dallo stato medio del pacco e la si scarica per p passi
% di controllo con la sola corrente di pacco, senza bilanciamento. La sua
% tensione a ogni passo e' il riferimento che le celle vere devono
% inseguire. Le grandezze della cella nominale hanno il suffisso 0, come
% l'apice 0 del paper: s0, Vp0, y0.
%
% Ingressi, misurati all'istante k
%   s, Vp     SOC e tensione di polarizzazione di ogni cella, N x 1
%   i_pacco   corrente di pacco [A], positiva in scarica
%   par_sim   parametri della simulazione (parametri_simulazione.m)
% Uscita
%   sigma0    riferimento, p x 1: la riga j vale per l'istante k+j
%
% Il modello della cella e' quello di Linearizzazione_MPC.pdf, citato [L]:
% equazioni (2), (3) e (4).

%% Dati
p     = par_sim.p;                      % passi dell'orizzonte
Tc    = par_sim.Tc;                     % [s] passo di controllo
kappa = par_sim.nominale.kappa;         % SOC perso in un passo per ogni ampere, [L, (5)]

% Tabelle della cella nominale: ogni parametro in 7 punti di SOC
s_tab   = par_sim.nominale.s_tab;
Voc_tab = par_sim.nominale.Voc_tab;     % [V]   tensione a vuoto
Ro_tab  = par_sim.nominale.Ro_tab;      % [Ohm] resistenza serie
Rp_tab  = par_sim.nominale.Rp_tab;      % [Ohm] resistenza di polarizzazione
Cp_tab  = par_sim.nominale.Cp_tab;      % [F]   capacita' di polarizzazione

%% Stato di partenza: la media delle celle del pacco
s0  = mean(s);
Vp0 = mean(Vp);

%% Scarica della cella nominale, un passo alla volta
sigma0 = zeros(p, 1);

for j = 1:p

    % Parametri del ramo RC nel SOC di inizio passo. Le tabelle vanno da
    % SOC 0 a SOC 1: fuori si usa il valore dell'estremo.
    s_limitato = min(max(s0, s_tab(1)), s_tab(end));
    Rp = interp1(s_tab, Rp_tab, s_limitato);
    Cp = interp1(s_tab, Cp_tab, s_limitato);

    % [L, (3)] tensione di polarizzazione a fine passo
    Vp0 = Vp0 + Tc * (-Vp0 / (Rp * Cp) + i_pacco / Cp);

    % [L, (2)] SOC a fine passo; una cella piena non si carica oltre
    s0 = s0 - kappa * i_pacco;
    if s0 > 1
        s0 = 1;
    end

    % [L, (4)] tensione ai morsetti a fine passo, con i parametri letti nel
    % nuovo SOC
    s_limitato = min(max(s0, s_tab(1)), s_tab(end));
    Voc = interp1(s_tab, Voc_tab, s_limitato);
    Ro  = interp1(s_tab, Ro_tab,  s_limitato);
    y0  = Voc - Vp0 - Ro * i_pacco;

    % Grandezza inseguita: la tensione, come nel paper, oppure il SOC
    if par_sim.sigma_tensione == 1
        sigma0(j) = y0;
    else
        sigma0(j) = s0;
    end

end

end

== matlab function Bilanciamento_MPC_2024b/Controllo/Problema_QP ==
  data: sigma0 input; H output; Y_bar input; S_bar input; d input; alfa input; u_bar input; f output; A output; b output; Aeq output; beq output; z_iniziale output; par_sim parameter
function [H, f, A, b, Aeq, beq, z_iniziale] = Problema_QP(sigma0, Y_bar, S_bar, d, alfa, u_bar, par_sim)
% PROBLEMA QP - il problema (6) del paper scritto come problema quadratico
% (Remark 3), nella forma che quadprog sa risolvere:
%
%   min  1/2*z'*H*z + f'*z     con  A*z <= b  e  Aeq*z = beq
%
% Il blocco non risolve nulla: riempie le matrici, un elemento alla volta,
% seguendo la procedura della sezione 8 di Problema_QP_MPC.pdf, citato [Q].
% I numeri come [Q, (12)] sono le equazioni di quel documento.
%
% Ingressi
%   sigma0         riferimento della cella nominale, p x 1 (serve solo a J_t)
%   Y_bar, S_bar   tensione e SOC predetti con u = u_bar, p x N
%   d, alfa        coefficienti di sensibilita' di tensione e SOC, p x N
%   u_bar          correnti di bilanciamento del passo precedente, N x 1
%   par_sim        parametri della simulazione (parametri_simulazione.m)
% Uscite
%   H, f, A, b, Aeq, beq   dati del QP
%   z_iniziale             punto di partenza ammissibile per quadprog
% Nelle matrici p x N la riga j corrisponde all'istante k+j, la colonna n
% alla cella n.

%% Dati
N     = par_sim.N;              % numero di celle
p     = par_sim.p;              % passi dell'orizzonte
n_J   = par_sim.n_J;            % formulazione: 1 = J_t, 2 = J_m, 3 = J_Delta
rho   = par_sim.rho;            % peso sulle correnti di bilanciamento
W     = par_sim.W;              % peso sulla variabile epsilon_y
y_min = par_sim.y_min;          % [V] tensione minima di cella
u_min = par_sim.u_min;          % [A] limiti della corrente di bilanciamento
u_max = par_sim.u_max;          % [A]

%% Incognite z = [u; epsilon; epsilon_y], [Q, sezione 8.1]
%   u(n)           corrente di bilanciamento della cella n     posizione n
%   epsilon(j)     minorante al passo j (J_m e J_Delta)        posizione N + j
%   epsilon(p+j)   maggiorante al passo j (solo J_Delta)       posizione N + p + j
%   epsilon_y      rilassamento della tensione minima          ultima posizione
n_z   = N + (n_J - 1) * p + 1;          % numero di incognite, [Q, (25)]
n_dis = n_J * p * N + 2 * N + 1;        % numero di vincoli di disuguaglianza, [Q, (25)]
pos_epsilon_y = n_z;                    % posizione di epsilon_y

%% Predizione linearizzata, [Q, (9)]
% Con la corrente u(n) la tensione predetta e'
%   y(j,n) = Y_lib(j,n) + d(j,n) * u(n)
% Y_lib e' la risposta libera: la tensione che si avrebbe senza bilanciamento.
Y_lib = zeros(p, N);
for n = 1:N
    for j = 1:p
        Y_lib(j, n) = Y_bar(j, n) - d(j, n) * u_bar(n);
    end
end

% Grandezza bilanciata sigma, usata dal costo e dai vincoli sulle epsilon:
% la tensione, come nel progetto, oppure il SOC ([Q, sezione 11]). Il
% vincolo di tensione minima usa sempre la tensione.
if par_sim.sigma_tensione == 1
    Sigma_bar = Y_bar;
    d_sigma   = d;
else
    Sigma_bar = S_bar;
    d_sigma   = alfa;
end
Sigma_lib = zeros(p, N);
for n = 1:N
    for j = 1:p
        Sigma_lib(j, n) = Sigma_bar(j, n) - d_sigma(j, n) * u_bar(n);
    end
end

%% Costruzione di H e di f, [Q, sezione 8.2]
H = zeros(n_z, n_z);
f = zeros(n_z, 1);

% Passo 1 - penalita' W*epsilon_y^2 (tutte le formulazioni), [Q, (13)]
H(pos_epsilon_y, pos_epsilon_y) = 2 * W;

% Passo 2 - peso rho*u(n)^2 sulle correnti (tutte le formulazioni), [Q, (14)]
for n = 1:N
    H(n, n) = 2 * rho;
end

% Passo 3 - inseguimento della cella nominale (solo J_t), [Q, (15)]
if n_J == 1
    for n = 1:N
        somma_d2 = 0;           % somma sui passi di d(j,n)^2
        somma_dc = 0;           % somma sui passi di d(j,n) * (Y_lib(j,n) - sigma0(j))
        for j = 1:p
            somma_d2 = somma_d2 + d_sigma(j, n)^2;
            somma_dc = somma_dc + d_sigma(j, n) * (Sigma_lib(j, n) - sigma0(j));
        end
        H(n, n) = H(n, n) + 2 * somma_d2;
        f(n)    = 2 * somma_dc;
    end
end

% Passo 4 - minoranti: nel costo -epsilon(j) (J_m e J_Delta), [Q, (18)]
if n_J == 2 || n_J == 3
    for j = 1:p
        f(N + j) = -1;
    end
end

% Passo 5 - maggioranti: nel costo +epsilon(p+j) (solo J_Delta), [Q, (21)]
if n_J == 3
    for j = 1:p
        f(N + p + j) = 1;
    end
end

%% Costruzione di A e di b, [Q, sezione 8.3]
% Ogni vincolo occupa una riga nuova: q e' il numero dell'ultima riga scritta.
A = zeros(n_dis, n_z);
b = zeros(n_dis, 1);
q = 0;

% Blocco 1 - tensione minima (tutte le formulazioni), [Q, (12)]:
%   -d(j,n)*u(n) - epsilon_y <= Y_lib(j,n) - y_min
for n = 1:N
    for j = 1:p
        q = q + 1;
        A(q, n)             = -d(j, n);
        A(q, pos_epsilon_y) = -1;
        b(q)                = Y_lib(j, n) - y_min;
    end
end

% Blocco 2 - minoranti (J_m e J_Delta), [Q, (17)]:
%   -d(j,n)*u(n) + epsilon(j) <= Y_lib(j,n)
if n_J == 2 || n_J == 3
    for n = 1:N
        for j = 1:p
            q = q + 1;
            A(q, n)     = -d_sigma(j, n);
            A(q, N + j) = 1;
            b(q)        = Sigma_lib(j, n);
        end
    end
end

% Blocco 3 - maggioranti (solo J_Delta), [Q, (20)]:
%   d(j,n)*u(n) - epsilon(p+j) <= -Y_lib(j,n)
if n_J == 3
    for n = 1:N
        for j = 1:p
            q = q + 1;
            A(q, n)         = d_sigma(j, n);
            A(q, N + p + j) = -1;
            b(q)            = -Sigma_lib(j, n);
        end
    end
end

% Blocco 4 - limite superiore delle correnti, [Q, (22)]:   u(n) <= u_max
for n = 1:N
    q = q + 1;
    A(q, n) = 1;
    b(q)    = u_max;
end

% Blocco 5 - limite inferiore delle correnti, [Q, (22)]:   -u(n) <= -u_min
for n = 1:N
    q = q + 1;
    A(q, n) = -1;
    b(q)    = -u_min;
end

% Blocco 6 - segno di epsilon_y, [Q, (23)]:   -epsilon_y <= 0
q = q + 1;
A(q, pos_epsilon_y) = -1;
b(q)                = 0;

%% Vincolo di uguaglianza: somma nulla delle correnti, [Q, (24)]
Aeq = zeros(1, n_z);
for n = 1:N
    Aeq(n) = 1;
end
beq = 0;

%% Punto di partenza, [Q, sezione 9, (26)]
% La mossa del passo precedente, completata con i valori delle epsilon che
% rispettano tutti i vincoli. Con u = u_bar la predizione vale Y_bar.
z_iniziale = zeros(n_z, 1);
for n = 1:N
    z_iniziale(n) = u_bar(n);
end
if n_J == 2 || n_J == 3
    for j = 1:p
        z_iniziale(N + j) = min(Sigma_bar(j, :));          % cella piu' bassa al passo j
    end
end
if n_J == 3
    for j = 1:p
        z_iniziale(N + p + j) = max(Sigma_bar(j, :));      % cella piu' alta al passo j
    end
end
z_iniziale(pos_epsilon_y) = max(0, y_min - min(Y_bar(:)));  % di quanto la predizione scende sotto y_min

end

== matlab function Bilanciamento_MPC_2024b/Controllo/Solutore_QP ==
  data: H input; u output; epsilon_y output; f input; A input; b input; Aeq input; beq input; z_iniziale input; esito output; par_sim parameter
function [u, epsilon_y, esito] = Solutore_QP(H, f, A, b, Aeq, beq, z_iniziale, par_sim)
% SOLUTORE QP - risolve il QP preparato dal blocco Problema_QP con quadprog,
% come nel paper (Sez. IV-A), e passa al pacco solo le correnti di
% bilanciamento (orizzonte mobile):
%
%   min  1/2*z'*H*z + f'*z     con  A*z <= b  e  Aeq*z = beq
%
% Uscite
%   u          prime N componenti di z: le correnti da applicare al passo k
%   epsilon_y  ultima componente di z: rilassamento del vincolo di tensione, eq. (17)
%   esito      exitflag di quadprog (1 = soluzione trovata)
%
% Se quadprog non trova una soluzione si usa z_iniziale, cioe' si mantiene
% la mossa del passo precedente, che rispetta sempre i vincoli.

% Opzioni del solutore, create al primo passo e poi conservate (persistent).
% Il metodo 'active-set' si ferma su un vertice esatto: adatto a J_m e
% J_Delta, che nelle variabili epsilon sono problemi lineari.
persistent opzioni
if isempty(opzioni)
    opzioni = optimoptions('quadprog', 'Algorithm', 'active-set', 'Display', 'off');
end

[z, ~, esito] = quadprog(H, f, A, b, Aeq, beq, [], [], z_iniziale, opzioni);

if esito <= 0 || isempty(z)
    z = z_iniziale;
end

u         = z(1:par_sim.N);
epsilon_y = z(end);

end
